simulink model "Battery_model_Hysterisis"  (R2025b)
settings: Solver=ode23  StartTime=0.0  StopTime=1000  MaxStep=0.01  RelTol=1e-4  AbsTol=1e-6
libraries: fl_lib x5, nesl_utility x5
settings Model: Creator=psvan  LastModifiedBy=psvan

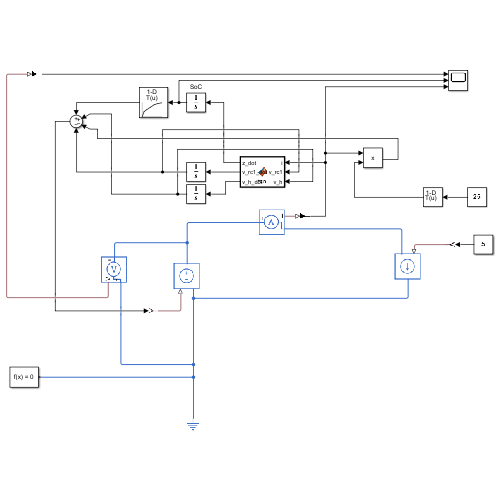
[thumbnail: Simulink's stored preview of the top-level diagram]
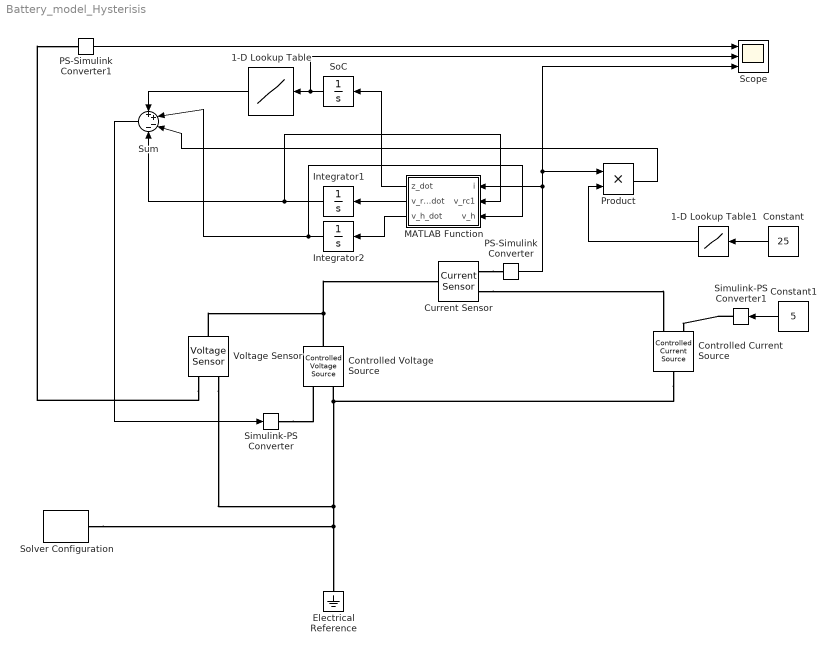
== system Battery_model_Hysterisis ==
  1-D Lookup Table : Lookup_n-D  NumberOfTableDimensions=1  BreakpointsForDimension1=[0,0.1,0.2,0.4,0.6,0.8,1.0]  Table=[3.0,3.4,3.6,3.8,4.0,4.1,4.2]  InternalRulePriority=Speed  RndMeth=Simplest
  1-D Lookup Table1 : Lookup_n-D  NumberOfTableDimensions=1  BreakpointsForDimension1=[0,25,40]  Table=[0.019,0.02,0.021]  InternalRulePriority=Speed  RndMeth=Simplest
  Constant : Constant  Value=25
  Constant1 : Constant  Value=5
  Controlled Current Source : fl_lib/Electrical/Electrical Sources/Controlled Current Source
  Controlled Voltage Source : fl_lib/Electrical/Electrical Sources/Controlled Voltage Source
  Current Sensor : fl_lib/Electrical/Electrical Sensors/Current Sensor
  Electrical Reference : fl_lib/Electrical/Electrical Elements/Electrical Reference
  Integrator1 : Integrator
  Integrator2 : Integrator
  MATLAB Function : MATLAB Function  TreatAsAtomicUnit=on
  PS-Simulink Converter : nesl_utility/PS-Simulink Converter  PhysicalDomain=network_engine_domain  SubClassName=ps_output  LeftPortType=input  RightPortType=output  PseudoPeriodic=off  Frequencies=[]  VectorFormat=inherit  Unit=inherit  AffineConversion=off
  PS-Simulink Converter1 : nesl_utility/PS-Simulink Converter  PhysicalDomain=network_engine_domain  SubClassName=ps_output  LeftPortType=input  RightPortType=output  PseudoPeriodic=off  Frequencies=[]  VectorFormat=inherit  Unit=inherit  AffineConversion=off
  Product : Product
  Scope : Scope  NumInputPorts=3
      settings: ActiveDisplayString=3  ActiveDisplayYMinimum=4  ActiveDisplayYMaximum=6  YLabel=Current
  Simulink-PS Converter : nesl_utility/Simulink-PS Converter  PhysicalDomain=network_engine_domain  SubClassName=ps_input  LeftPortType=input  RightPortType=output  PseudoPeriodic=off  Frequencies=[]  NoiseDistribution=none  NoiseParameters=[]  Unit=1  AffineConversion=off  FilteringAndDerivatives=provide  SimscapeFilterOrder=1  InputFilterTimeConstant=0.001  UdotUserProvided=0
  Simulink-PS Converter1 : nesl_utility/Simulink-PS Converter  PhysicalDomain=network_engine_domain  SubClassName=ps_input  LeftPortType=input  RightPortType=output  PseudoPeriodic=off  Frequencies=[]  NoiseDistribution=none  NoiseParameters=[]  Unit=1  AffineConversion=off  FilteringAndDerivatives=provide  SimscapeFilterOrder=1  InputFilterTimeConstant=0.001  UdotUserProvided=0
  SoC : Integrator  InitialCondition=0.5
  Solver Configuration : nesl_utility/Solver Configuration  PhysicalDomain=network_engine_domain  SubClassName=solver  LeftPortType=input  RightPortType=generic  Tones=[]  Harmonics=[]  SimulateNoise=off  Profile=off  UseLocalSampling=off  EnableSwitchedLinearOptims=on  FrequencyDomain=off  UseCCode=off  RelTol=0.001  AbsTol=0.001  MinStep=1e-09  ToWorkspace=off  RevertToSquareIcSolve=off  NumHomotopyIterations=100  PhasorMode=off  PhasorModeNumHarmonics=1  ConsistencySolver=NEWTON_XTOL_AFTER_FTOL  IndexReductionMethod=DerivativeReplacement  DoDC=off  ResidualTolerance=1e-09  ConsistencyTolSource=GLOBAL  ConsistencyAbsTol=0.001  ConsistencyRelTol=0.001  ConsistencyTolFactor=0.001  UseLocalSolver=off  LocalSolverChoice=NE_BACKWARD_EULER_ADVANCER  ResolveIndetEquations=on  FunctionEvalNumThread=1  LocalSolverSampleTime=0.001  DoFixedCost=off  MaxNonlinIter=3  MaxModeIter=2  ComputeImpulses=off  ImpulseIterations=2  LinearAlgebra=auto  LinearAlgebraNumThread=0  EquationFormulation=NE_TIME_EF  DelaysMemoryBudget=1024  AutomaticFiltering=on  FilteringTimeConstant=0.001  PartitionStorageMethod=AS_NEEDED  PartitionMemoryBudget=1024  PartitionMethod=ROBUST  MultibodyUseLocalSolver=off  MultibodyLocalSolverChoice=ODE1  MultibodyLocalSolverSampleTime=0.001
  Sum : Sum  Inputs=++--
  Voltage Sensor : fl_lib/Electrical/Electrical Sensors/Voltage Sensor
  wires:
  PS-Simulink Converter/1 -> Scope/3, Product/1, MATLAB Function/1(i)
  MATLAB Function/1(z_dot) -> SoC/1
  MATLAB Function/2(v_rc1_dot) -> Integrator1/1
  Integrator1/1 -> MATLAB Function/2(v_rc1), Sum/4
  MATLAB Function/3(v_h_dot) -> Integrator2/1
  Integrator2/1 -> Sum/2, MATLAB Function/3(v_h)
  SoC/1 -> Scope/2, 1-D Lookup Table/1
  Constant/1 -> 1-D Lookup Table1/1
  1-D Lookup Table1/1 -> Product/2
  1-D Lookup Table/1 -> Sum/1
  Product/1 -> Sum/3
  Sum/1 -> Simulink-PS Converter/1
  Constant1/1 -> Simulink-PS Converter1/1
  PS-Simulink Converter1/1 -> Scope/1
  connections:
  Controlled Current Source/LConn1 -- Voltage Sensor/RConn2 -- Solver Configuration/RConn1 -- Electrical Reference/LConn1 -- Controlled Voltage Source/RConn2
  Controlled Voltage Source/LConn1 -- Voltage Sensor/LConn1 -- Current Sensor/LConn1
  Current Sensor/RConn2 -- Controlled Current Source/RConn2
  Current Sensor/RConn1 -- PS-Simulink Converter/LConn1
  Simulink-PS Converter/RConn1 -- Controlled Voltage Source/RConn1
  Simulink-PS Converter1/RConn1 -- Controlled Current Source/RConn1
  Voltage Sensor/RConn1 -- PS-Simulink Converter1/LConn1

== matlab function Battery_model_Hysterisis/MATLAB Function ==
  data: i input; z_dot output; v_rc1 input; v_h input; v_rc1_dot output; v_h_dot output
function [z_dot, v_rc1_dot, v_h_dot] = fcn(i, v_rc1, v_h)


Q = 3600;      
eta = 0.995;   
R1 = 0.01;     
C1 = 500;     
M = 0.05;      
gamma = 10;    

z_dot = -(eta * i) / Q;

v_rc1_dot = (i / C1) - (v_rc1 / (R1 * C1));

current_sign = 1; 
if i < 0
    current_sign = -1; 
end

v_h_dot = gamma * abs(i) * (M * current_sign - v_h);

end
